simulink model "controle_pi"  (R2025a)
settings: Solver=FixedStepAuto  StartTime=0.0  StopTime=0.2  FixedStep=1e-6  RelTol=1e-3
values from neighbouring files (symbols this model uses):
  Ki = 400    [projeto_pi.m]
  Kp = 10    [projeto_pi.m]
  L = 0.01    [projeto_pi.m]
  R = 4    [projeto_pi.m]
  Wt = 2*pi*60    (= 376.991118431)    [projeto_pi.m]
libraries: spsSeriesRLCBranchLib x5, spsDCVoltageSourceLib x1, spsAlphaBetaZerotoabcLib x1, spsAlphaBetaZerotodq0Lib x1, spsGroundLib x1, eePwmGeneratorTwoLevel x1, spsThreePhaseVIMeasurementLib x1, spsUniversalBridgeLib x1, spsabctoAlphaBetaZeroLib x1, spsdq0toAlphaBetaZeroLib x1, sps_lib x1
settings Model: Creator=Alessandra Costa  LastModifiedBy=raphateixeira

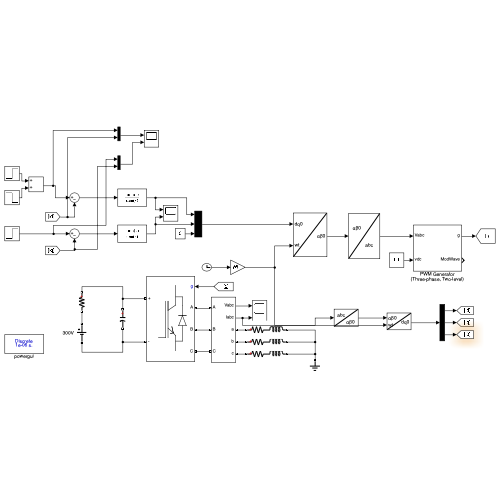
[thumbnail: Simulink's stored preview of the top-level diagram]
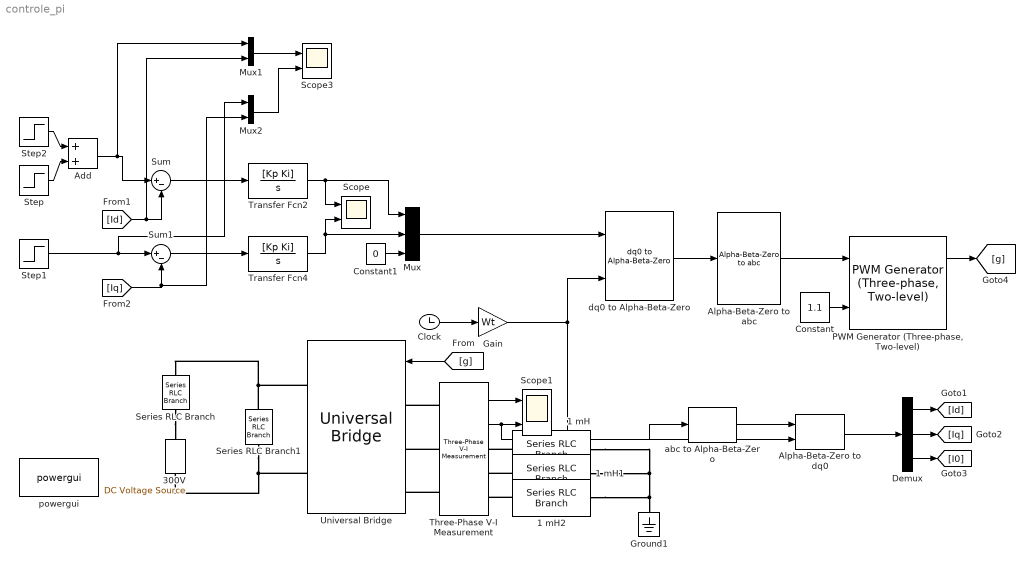
== system controle_pi ==
  1 mH : spsSeriesRLCBranchLib/Series RLC Branch  LConnTagsString=__new0  RConnTagsString=__new0  BranchType=RL  Resistance=R  Inductance=L  SetiL0=off  InitialCurrent=0  Capacitance=1e-6  Setx0=off  InitialVoltage=0  Measurements=None
  1 mH1 : spsSeriesRLCBranchLib/Series RLC Branch  LConnTagsString=__new0  RConnTagsString=__new0  BranchType=RL  Resistance=R  Inductance=L  SetiL0=off  InitialCurrent=0  Capacitance=1e-6  Setx0=off  InitialVoltage=0  Measurements=None
  1 mH2 : spsSeriesRLCBranchLib/Series RLC Branch  LConnTagsString=__new0  RConnTagsString=__new0  BranchType=RL  Resistance=R  Inductance=L  SetiL0=off  InitialCurrent=0  Capacitance=1e-6  Setx0=off  InitialVoltage=0  Measurements=None
  300V : spsDCVoltageSourceLib/DC Voltage Source  Amplitude=300  Measurements=None
  Add : Sum
  Alpha-Beta-Zero to abc : spsAlphaBetaZerotoabcLib/Alpha-Beta-Zero to abc
      settings: LibrarySourceBlock=|
      | sps_lib/Control/Alpha-Beta-Zero
      | to abc
  Alpha-Beta-Zero to dq0 : spsAlphaBetaZerotodq0Lib/Alpha-Beta-Zero to dq0  Alignment=90 degrees behind phase A axis
  Clock : Clock
  Constant : Constant  Value=1.1
  Constant1 : Constant  Value=0
  Demux : Demux  Outputs=3
  Gain : Gain  Gain=Wt
  Ground1 : spsGroundLib/Ground  LConnTagsString=a
  Mux : Mux  Inputs=3
  Mux1 : Mux  Inputs=2
  Mux2 : Mux  Inputs=2
  "PWM Generator (Three-phase, Two-level)" : eePwmGeneratorTwoLevel/PWM Generator (Three-phase, Two-level)  PWMMode=Continuous PWM (CPWM)  CPWMMode=SPWM: sinusoidal PWM  DPWMMode=60 DPWM: 60 degree discontinuous PWM  fsw=10000  Ts=1e-6
      settings: LibrarySourceBlock=|
      | ee_sl_lib/Pulse Width
      | Modulation/PWM Generator
      | (Three-phase, Two-level)
  Scope : Scope  NumInputPorts=2
      settings: ActiveDisplayYMinimum=-14.884466195650347  ActiveDisplayYMaximum=34.987162910627816
  Scope1 : Scope  NumInputPorts=2
      settings: ActiveDisplayYMinimum=-8.37511  ActiveDisplayYMaximum=7.91214
  Scope3 : Scope  NumInputPorts=2
      settings: ActiveDisplayYMinimum=1.8394309188386511  ActiveDisplayYMaximum=3.0544731303141539  DataLoggingVariableName=ScopeData3
  Series RLC Branch : spsSeriesRLCBranchLib/Series RLC Branch  LConnTagsString=__new0  RConnTagsString=__new0  BranchType=R  Resistance=R  Inductance=1e-3  SetiL0=off  InitialCurrent=0  Capacitance=1e-6  Setx0=off  InitialVoltage=0  Measurements=None
  Series RLC Branch1 : spsSeriesRLCBranchLib/Series RLC Branch  LConnTagsString=__new0  RConnTagsString=__new0  BranchType=C  Resistance=0.1  Inductance=1e-3  SetiL0=off  InitialCurrent=0  Capacitance=1000e-6  Setx0=off  InitialVoltage=0  Measurements=None
  Step : Step  Time=0.1  After=-1  SampleTime=0
  Step1 : Step  Time=0  After=3  SampleTime=0
  Step2 : Step  Time=0  After=3  SampleTime=0
  Sum : Sum  Inputs=|+-
  Sum1 : Sum  Inputs=|+-
  Three-Phase V-I Measurement : spsThreePhaseVIMeasurementLib/Three-Phase V-I Measurement  VoltageMeasurement=phase-to-ground  SetLabelV=off  LabelV=Vabc  Vpu=off  VpuLL=off  CurrentMeasurement=yes  SetLabelI=off  LabelI=Iabc  Ipu=off  Pbase=100e6  Vbase=500e3  OutputType=Complex  PhasorSimulation=off  PSBequivalent=0
  Transfer Fcn2 : TransferFcn  Numerator=[Kp Ki]  Denominator=[1 0]
  Transfer Fcn4 : TransferFcn  Numerator=[Kp Ki]  Denominator=[1 0]
  Universal Bridge : spsUniversalBridgeLib/Universal Bridge  Arms=3  SnubberResistance=1e5  SnubberCapacitance=inf  Device=IGBT / Diodes  Ron=1e-3  Lon=0  ForwardVoltages="[  0  0  ]"  ForwardVoltage=0  GTOparameters=[ 10e-6 , 20e-6 ]  IGBTparameters=[ 1e-6 , 2e-6 ]  Measurements=None  Measurements_2=None  converterType=Rectifier
  abc to Alpha-Beta-Zero : spsabctoAlphaBetaZeroLib/abc to Alpha-Beta-Zero
  dq0 to Alpha-Beta-Zero : spsdq0toAlphaBetaZeroLib/dq0 to Alpha-Beta-Zero  Alignment=90 degrees behind phase A axis
  powergui : sps_lib/powergui  Priority=1  SimulationMode=Discrete  SampleTime=1e-6  frequency=60  Iterations=50  frequencyindice=0  Pbase=100e6  ErrMax=1e-4  UnitsV=kV  UnitsW=MW  buscounter=0  FunctionMessages=off  echomessages=off  EnableUseOfTLC=off  CurrentSourceSwitches=off  DisableSnubberDevices=off  DisableRonSwitches=off  DisableVfSwitches=off  DisplayEquations=off  AutomaticDiscreteSolvers=off  SolverType=Tustin/Backward Euler (TBE)  Interpol=off  ExternalGateDelay=off  methode=off  Ts=100  x0status=blocks  SPID=on  SwTol=0  HookPort=off  NonlinearTolerance=1e-4  nMaxIteration=100  ContinueOnMaxIteration=off  RestoreLinks=warning  ResistiveCurrentMeasurement=off  Frange=[0:2:500]  Ylog=off  Xlog=on  ShowGrid=off  save=off  variable=ZData  structure=0  ZoomFFT=off  StartTime=0.0  cycles=1  DisplayStyle=1  fundamental=60  FreqAxis=off  MaxFrequency=1000  frequencyindicesteady=1  RmsSteady=1  display=off
  wires:
  Constant/1 -> "PWM Generator (Three-phase, Two-level)"/2
  Step1/1 -> Mux2/1, Sum1/1
  Transfer Fcn2/1 -> Mux/1, Scope/1
  Sum/1 -> Transfer Fcn2/1
  Sum1/1 -> Transfer Fcn4/1
  dq0 to Alpha-Beta-Zero/1 -> Alpha-Beta-Zero to abc/1
  Alpha-Beta-Zero to abc/1 -> "PWM Generator (Three-phase, Two-level)"/1
  abc to Alpha-Beta-Zero/1 -> Alpha-Beta-Zero to dq0/1
  Transfer Fcn4/1 -> Mux/2, Scope/2
  Mux/1 -> dq0 to Alpha-Beta-Zero/1
  Clock/1 -> Gain/1
  "PWM Generator (Three-phase, Two-level)"/1 -> [g]
  [g] -> Universal Bridge/1
  Alpha-Beta-Zero to dq0/1 -> Demux/1
  Demux/1 -> [Id]
  Demux/2 -> [Iq]
  [Id] -> Mux1/2, Sum/2
  [Iq] -> Mux2/2, Sum1/2
  Constant1/1 -> Mux/3
  Demux/3 -> [I0]
  Gain/1 -> Alpha-Beta-Zero to dq0/2, dq0 to Alpha-Beta-Zero/2
  Mux1/1 -> Scope3/1
  Mux2/1 -> Scope3/2
  Step2/1 -> Add/1
  Step/1 -> Add/2
  Add/1 -> Mux1/1, Sum/1
  Three-Phase V-I Measurement/1 -> Scope1/1
  Three-Phase V-I Measurement/2 -> abc to Alpha-Beta-Zero/1, Scope1/2
  connections:
  Universal Bridge/RConn1 -- Series RLC Branch1/LConn1 -- Series RLC Branch/LConn1
  Series RLC Branch1/RConn1 -- Universal Bridge/RConn2 -- 300V/LConn1
  Series RLC Branch/RConn1 -- 300V/RConn1
  Three-Phase V-I Measurement/LConn1 -- Universal Bridge/LConn1
  Three-Phase V-I Measurement/LConn2 -- Universal Bridge/LConn2
  Three-Phase V-I Measurement/LConn3 -- Universal Bridge/LConn3
  1 mH/LConn1 -- Three-Phase V-I Measurement/RConn1
  1 mH1/LConn1 -- Three-Phase V-I Measurement/RConn2
  1 mH2/LConn1 -- Three-Phase V-I Measurement/RConn3
  1 mH/RConn1 -- 1 mH1/RConn1 -- 1 mH2/RConn1 -- Ground1/LConn1
